simulink model "simulacija_odredjivanje_parametara"  (R2015b)
settings: Solver=FixedStepAuto  StartTime=0.0  StopTime=20  FixedStep=0.001  RelTol=1e-3
libraries: simulink x1
settings Model: Creator=admin  LastModifiedBy=Elma

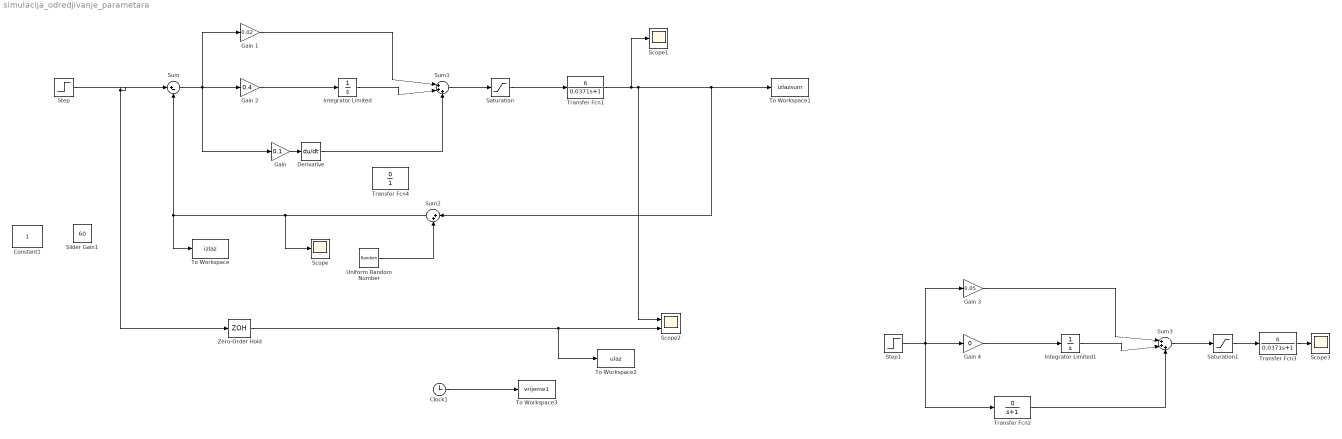
== system simulacija_odredjivanje_parametara ==
  Clock1 : Clock
  Constant1 : Constant
  Derivative : Derivative
  Gain : Gain  Gain=0.1
  Gain 1 : Gain  Gain=0.02
  Gain 2 : Gain  Gain=0.4
  Gain 3 : Gain  Gain=0.05
  Gain 4 : Gain  Gain=0
  Integrator Limited : Integrator  LimitOutput=on  UpperSaturationLimit=10  LowerSaturationLimit=0
  Integrator Limited1 : Integrator  LimitOutput=on  UpperSaturationLimit=10  LowerSaturationLimit=0
  Saturation : Saturate  UpperLimit=10  LowerLimit=0
  Saturation1 : Saturate  UpperLimit=10  LowerLimit=0
  Scope : Scope
  Scope1 : Scope
  Scope2 : Scope  NumInputPorts=2
  Scope3 : Scope
  Slider Gain1 : simulink/Math Operations/Slider Gain  low=0  gain=60  high=60
  Step : Step  After=60  SampleTime=0
  Step1 : Step  SampleTime=0
  Sum : Sum  Inputs=|+-
  Sum1 : Sum  Inputs=|+++
  Sum2 : Sum  Inputs=|++
  Sum3 : Sum  Inputs=|+++
  To Workspace : ToWorkspace  VariableName=izlaz  SampleTime=-1
      settings: Save2DSignal=2-D array (concatenate along first dimension)
  To Workspace1 : ToWorkspace  VariableName=izlazsum  SampleTime=-1
      settings: Save2DSignal=2-D array (concatenate along first dimension)
  To Workspace2 : ToWorkspace  VariableName=ulaz  SampleTime=-1
  To Workspace3 : ToWorkspace  VariableName=vrijeme1  SampleTime=-1
      settings: Save2DSignal=2-D array (concatenate along first dimension)
  Transfer Fcn1 : TransferFcn  Numerator=[6]  Denominator=[0.0371 1]
  Transfer Fcn2 : TransferFcn  Numerator=[0 0]  Denominator=[1 1]
  Transfer Fcn3 : TransferFcn  Numerator=[6]  Denominator=[0.0371 1]
  Transfer Fcn4 : TransferFcn  Numerator=[0 0]  Denominator=[0.0000 1]
  Uniform Random Number : UniformRandomNumber  Minimum=0  Maximum=0.2  SampleTime=0.001
  Zero-Order Hold : ZeroOrderHold  SampleTime=0.001
  wires:
  Step/1 -> Sum/1, Zero-Order Hold/1
  Sum/1 -> Gain/1, Gain 1/1, Gain 2/1
  Gain 1/1 -> Sum1/1
  Integrator Limited/1 -> Sum1/2
  Derivative/1 -> Sum1/3
  Sum1/1 -> Saturation/1
  Saturation/1 -> Transfer Fcn1/1
  Transfer Fcn1/1 -> Scope1/1, Scope2/1, Sum2/1, To Workspace1/1
  Uniform Random Number/1 -> Sum2/2
  Sum2/1 -> Scope/1, To Workspace/1, Sum/2
  Gain 2/1 -> Integrator Limited/1
  Zero-Order Hold/1 -> To Workspace2/1, Scope2/2
  Clock1/1 -> To Workspace3/1
  Step1/1 -> Transfer Fcn2/1, Gain 3/1, Gain 4/1
  Gain 3/1 -> Sum3/1
  Integrator Limited1/1 -> Sum3/2
  Transfer Fcn2/1 -> Sum3/3
  Sum3/1 -> Saturation1/1
  Saturation1/1 -> Transfer Fcn3/1
  Gain 4/1 -> Integrator Limited1/1
  Transfer Fcn3/1 -> Scope3/1
  Gain/1 -> Derivative/1
